simulink model "p88_stop_sign_detector"  (R2026a)
settings: Solver=ode3  StopTime=inf  EnableMultiTasking=on
StopFcn:
  | h=findobj('type','figure');if ~isempty(h);close(h); clear h; end
model workspace (MAT data in the model file):
  RGB_image = [255 255 255 255 255 255 255 255 255 255 255 255 ... (230400 elements, 240x320x3)]
libraries: raspberrypiAVlib x2
(part 1 of 2)
settings Model: FPTRunName=Active  ExtModeTrigDuration=2  Creator=The MathWorks, Inc.  LastModifiedBy=User
settings SolverCC: PositivePriorityOrder=on
settings OptimizationCC: LifeSpan=Inf  MaxStackSize=200000
settings HardwareCC: ProdBitPerLong=64.0  ProdLargestAtomicInteger=LongLong  ProdLargestAtomicFloat=Double  ProdHWDeviceType=ARM Compatible->ARM Cortex-A (64-bit)
settings RTWCC: SystemTargetFile=ert.tlc  HardwareBoard=Raspberry Pi (64bit)  TLCOptions="-aInlineSetEventsForThisBaseRateFcn=TLC_FALSE -aSuppressMultiTaskScheduler=TLC_FALSE  -aRateBasedStepFcn=0"  Toolchain=GNU GCC RPIUtils  BuildConfiguration=Faster Runs  DLArmComputeArch=armv7  Description=Embedded Coder
settings ERTTargetCC: ExtModeTransport=2.0  DynamicArrayContainerType=coder::array  MultiwordLength=2048.0  ERTCustomFileBanners=off  SupportContinuousTime=on  SupportNonInlinedSFcns=on  SupportVariableSizeSignals=on  ModelStepFunctionPrototypeControlCompliant=off

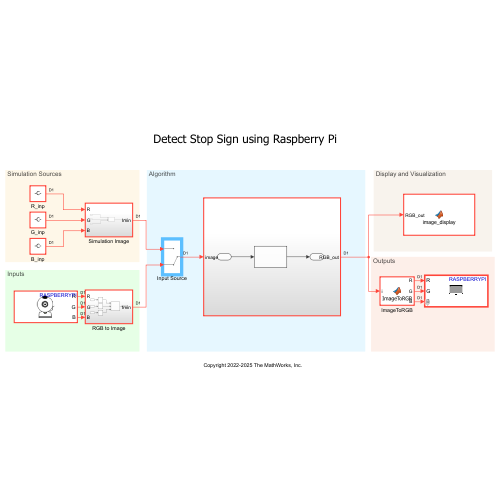
[thumbnail: Simulink's stored preview of the top-level diagram]
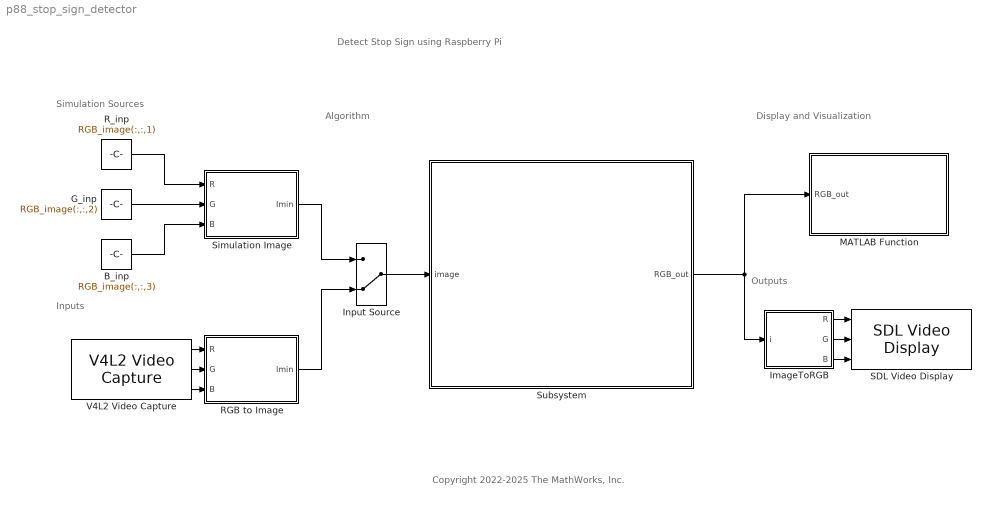
== system p88_stop_sign_detector ==
  note: Display and Visualization
  note: Outputs
  note: Simulation Sources
  note: Detect Stop Sign using Raspberry Pi
  note: Algorithm
  note: Inputs
  note: Copyright 2022-2025 The MathWorks, Inc.
  B_inp : Constant  Value=RGB_image(:,:,3)  OutDataTypeStr=uint8  SampleTime=0.1
  G_inp : Constant  Value=RGB_image(:,:,2)  OutDataTypeStr=uint8  SampleTime=0.1
  ImageToRGB : MATLAB Function  TreatAsAtomicUnit=on
  Input Source : ManualSwitch  CurrentSetting=0
  MATLAB Function : MATLAB Function  TreatAsAtomicUnit=on
  RGB to Image : Subsystem
  R_inp : Constant  Value=RGB_image(:,:,1)  OutDataTypeStr=uint8  SampleTime=0.1
  SDL Video Display : raspberrypiAVlib/SDL Video Display  title=SDL Video Display  pixelFormat=RGB  pixelOrder=Planar  rowMajor=on  blockPlatform=Raspberry Pi
  Simulation Image : Subsystem
  Subsystem : Subsystem
  V4L2 Video Capture : raspberrypiAVlib/V4L2 Video Capture  DeviceName=/dev/video0  Resolution=320x240  CustomResolution=[ 320, 240 ]  PixelFormat=RGB  SampleTime=0.1  pixelOrder=planar  simOutput=Colorbars  imSizeSelection=320x240  imSize=[640, 480]  roi=[0, 0, 640, 480]  m_devName='/dev/video0'  blockPlatform=LINUX  HorizontalFlip=off  VerticalFlip=off  Brightness=0.5  Saturation=0.5  Contrast=0.5  Sharpness=0.5  CameraPan=0  CameraTilt=0  CameraZoom=0.5  EnableManualFocus=on  ManualFocus=0.5
  wires:
  V4L2 Video Capture/1 -> RGB to Image/1(R)
  V4L2 Video Capture/2 -> RGB to Image/2(G)
  V4L2 Video Capture/3 -> RGB to Image/3(B)
  R_inp/1 -> Simulation Image/1(R)
  G_inp/1 -> Simulation Image/2(G)
  B_inp/1 -> Simulation Image/3(B)
  Input Source/1 -> Subsystem/1(image)
  Simulation Image/1(Imin) -> Input Source/1
  RGB to Image/1(Imin) -> Input Source/2
  ImageToRGB/1(R) -> SDL Video Display/1
  ImageToRGB/2(G) -> SDL Video Display/2
  ImageToRGB/3(B) -> SDL Video Display/3
  Subsystem/1(RGB_out) -> ImageToRGB/1(i), MATLAB Function/1(RGB_out)
